simulink model "Response_Animations"  (R2025b)
settings: Solver=VariableStepAuto  StartTime=0.0  StopTime=15  RelTol=1e-3
libraries: simulink_extras x4, aerolibanim x2
settings Model: Creator=maxma  LastModifiedBy=maxma

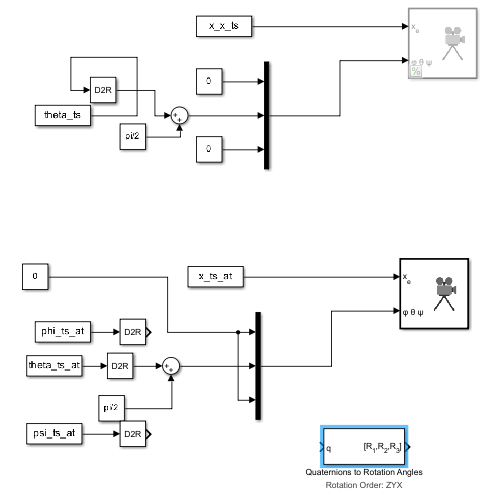
[thumbnail: Simulink's stored preview of the top-level diagram]
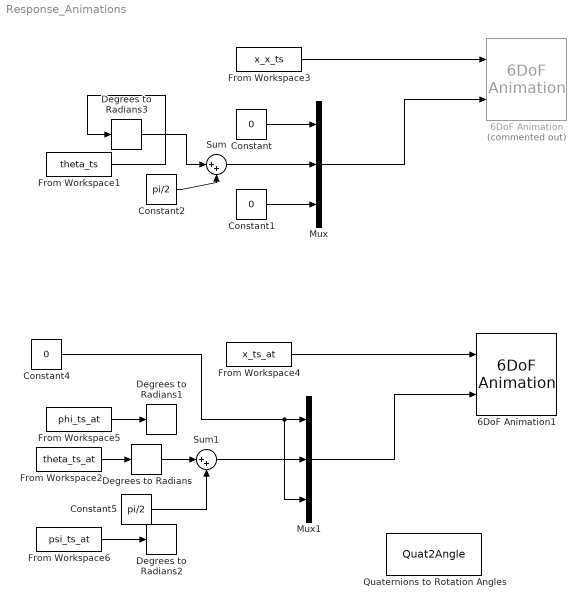
== system Response_Animations ==
  6DoF Animation : aerolibanim/6DoF Animation  Commented=on  u1=[-10 10 -10 10 -10 10]  u2=0.1  u3=1  u4=[4000 0 -5000]  u5=Fixed position  u6=[10 -10 0]  u7=5  u8=on
  6DoF Animation1 : aerolibanim/6DoF Animation  u1=[-10 10 -10 10 -10 10]  u2=0.1  u3=1  u4=[4000 0 -5000]  u5=Fixed position  u6=[10 -10 0]  u7=5  u8=on
  Constant : Constant  Value=0
  Constant1 : Constant  Value=0
  Constant2 : Constant  Value=pi/2
  Constant4 : Constant  Value=0
  Constant5 : Constant  Value=pi/2
  Degrees to Radians{,1..3} (4 alike) : simulink_extras/Transformations/Degrees to Radians
  From Workspace1 : FromWorkspace  VariableName=theta_ts
  From Workspace2 : FromWorkspace  VariableName=theta_ts_at
  From Workspace3 : FromWorkspace  VariableName=x_x_ts
  From Workspace4 : FromWorkspace  VariableName=x_ts_at
  From Workspace5 : FromWorkspace  VariableName=phi_ts_at
  From Workspace6 : FromWorkspace  VariableName=psi_ts_at
  Mux : Mux  Inputs=3
  Mux1 : Mux  Inputs=3
  Quaternions to Rotation Angles : Quat2Angle
      settings: AttributesFormatString=Rotation Order: %<rotationOrder>
  Sum : Sum  Inputs=|++
  Sum1 : Sum  Inputs=|++
  wires:
  Mux/1 -> 6DoF Animation/2
  From Workspace3/1 -> 6DoF Animation/1
  Constant/1 -> Mux/1
  Constant1/1 -> Mux/3
  Sum/1 -> Mux/2
  Constant2/1 -> Sum/2
  Sum1/1 -> Mux1/2
  Mux1/1 -> 6DoF Animation1/2
  From Workspace4/1 -> 6DoF Animation1/1
  Degrees to Radians/1 -> Sum1/1
  From Workspace2/1 -> Degrees to Radians/1
  Constant5/1 -> Sum1/2
  From Workspace5/1 -> Degrees to Radians1/1
  From Workspace6/1 -> Degrees to Radians2/1
  From Workspace1/1 -> Degrees to Radians3/1
  Degrees to Radians3/1 -> Sum/1
  Constant4/1 -> Mux1/3, Mux1/1
